simulink model "Fig330L1_THD5_tuned_gridRC2_2wai"  (R2021b)
settings: Solver=ode45  StartTime=0.0  StopTime=0.3  RelTol=1e-3
libraries: spsSeriesRLCBranchLib x17, spsThreePhaseVIMeasurementLib x6, spsIGBTDiodeLib x6, spsGroundLib x4, eePowerMeasurement x4, spsVoltageMeasurementLib x4, spsSecondOrderFilterLib x2, spsabctoAlphaBetaZeroLib x2, spsabctodq0Lib x2, spsDCVoltageSourceLib x1, simulink x1, spsThreePhaseProgrammableVoltageSourceLib x1
settings Model: Creator=cym1999  LastModifiedBy=caoyanmin
settings DataIOCC: ReturnWorkspaceOutputs=off

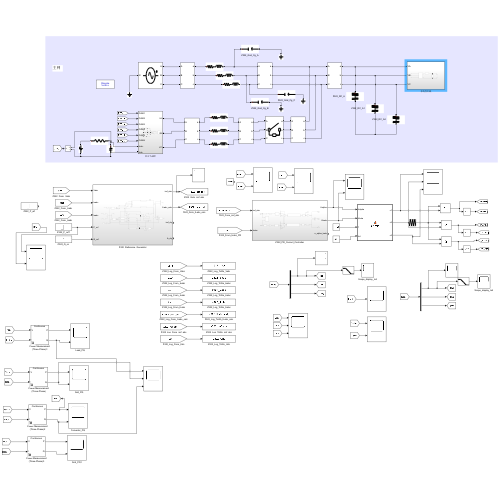
[thumbnail: Simulink's stored preview of the top-level diagram]
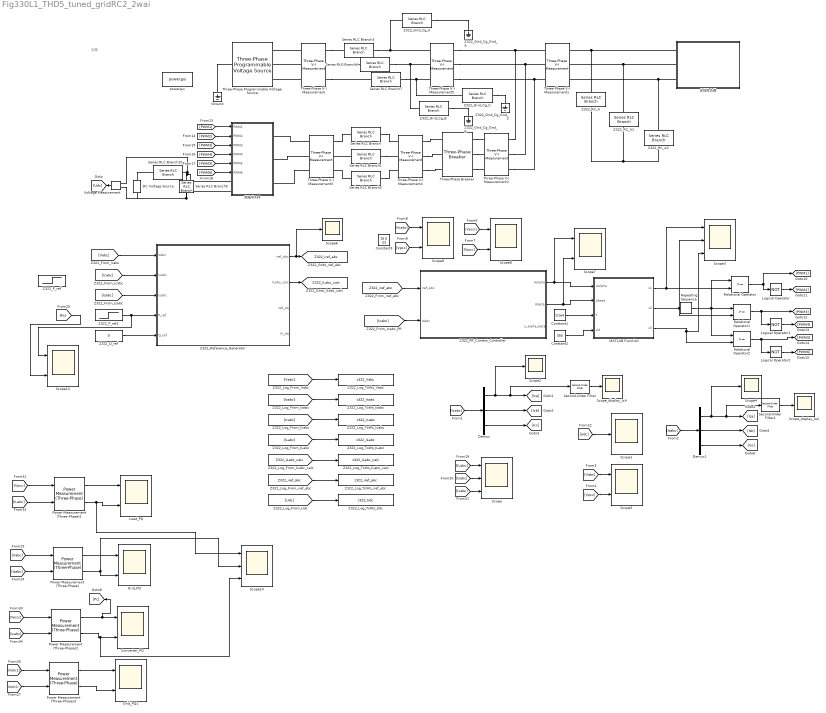
== system Fig330L1_THD5_tuned_gridRC2_2wai ==
  note: 主网
  Constant1 : Constant  Value=1/1e4
  Constant2 : Constant  Value=350
  Constant3 : Constant  Value=[0 0 0]
  Converter_PQ : Scope  NumInputPorts=2
  DC Voltage Source : spsDCVoltageSourceLib/DC Voltage Source  Amplitude=350  Measurements=None
  Demux : Demux  Outputs=3
  Demux1 : Demux  Outputs=3
  Grid_PQ : Scope  NumInputPorts=2
  Grid_PQ1 : Scope  NumInputPorts=2
  Ground : spsGroundLib/Ground  LConnTagsString=a
  Load_PQ : Scope  NumInputPorts=2
  Logical Operator : Logic  Operator=NOT  Inputs=1  AllPortsSameDT=off  OutDataTypeStr=boolean
  Logical Operator1 : Logic  Operator=NOT  Inputs=1  AllPortsSameDT=off  OutDataTypeStr=boolean
  Logical Operator2 : Logic  Operator=NOT  Inputs=1  AllPortsSameDT=off  OutDataTypeStr=boolean
  MATLAB Function : MATLAB Function  TreatAsAtomicUnit=on
  Power Measurement (Three-Phase){,1..3} (4 alike) : eePowerMeasurement/Power Measurement (Three-Phase)  LabelModeActiveChoice=Continuous  F=50  K=[1]  Seq=Positive  Ts=0
      settings: SourceProductBaseCode=PS
  Relational Operator : RelationalOperator  OutDataTypeStr=boolean  RndMeth=Simplest
  Relational Operator1 : RelationalOperator  OutDataTypeStr=boolean  RndMeth=Simplest
  Relational Operator2 : RelationalOperator  OutDataTypeStr=boolean  RndMeth=Simplest
  Repeating Sequence : simulink/Sources/Repeating Sequence  rep_seq_t=[0 0.00005 0.0001]  rep_seq_y=[0 0.0001/2 0]
  Scope : Scope  NumInputPorts=3
  Scope{1..2,4,6} (4 alike) : Scope
  Scope{5,7..9,13} (5 alike) : Scope  NumInputPorts=2
  Scope14 : Scope  NumInputPorts=3
  Scope3 : Scope  NumInputPorts=3
  Scope_display_IcA : Scope
  Scope_display_IsA : Scope
  Second-Order Filter : spsSecondOrderFilterLib/Second-Order Filter  FilterType=Lowpass  Fo=1000  Zeta=0.707  Ts=1e-6  Initialize=on  Vac_Init="[0,  0,  60]"  Vdc_Init=0  PlotResponse=off  FreqRange=[0, 500, 1]
      settings: SourceProductBaseCode=PS
  Second-Order Filter1 : spsSecondOrderFilterLib/Second-Order Filter  FilterType=Lowpass  Fo=1000  Zeta=0.707  Ts=1e-6  Initialize=on  Vac_Init="[0,  0,  60]"  Vdc_Init=0  PlotResponse=off  FreqRange=[0, 500, 1]
      settings: SourceProductBaseCode=PS
  Series RLC Branch : spsSeriesRLCBranchLib/Series RLC Branch  LConnTagsString=__new0  RConnTagsString=__new0  BranchType=RL  Resistance=0.05  Inductance=5e-4  SetiL0=off  InitialCurrent=0  Capacitance=1e-6  Setx0=off  InitialVoltage=0  Measurements=None
  Series RLC Branch1 : spsSeriesRLCBranchLib/Series RLC Branch  LConnTagsString=__new0  RConnTagsString=__new0  BranchType=RL  Resistance=0.05  Inductance=5e-4  SetiL0=off  InitialCurrent=0  Capacitance=1e-6  Setx0=off  InitialVoltage=0  Measurements=None
  Series RLC Branch10 : spsSeriesRLCBranchLib/Series RLC Branch  LConnTagsString=__new0  RConnTagsString=__new0  BranchType=R  Resistance=0.01  Inductance=2.56e-3  SetiL0=off  InitialCurrent=0  Capacitance=1e-6  Setx0=off  InitialVoltage=0  Measurements=None
  Series RLC Branch2 : spsSeriesRLCBranchLib/Series RLC Branch  LConnTagsString=__new0  RConnTagsString=__new0  BranchType=RL  Resistance=0.05  Inductance=5e-4  SetiL0=off  InitialCurrent=0  Capacitance=1e-6  Setx0=off  InitialVoltage=0  Measurements=None
  Series RLC Branch3 : spsSeriesRLCBranchLib/Series RLC Branch  LConnTagsString=__new0  RConnTagsString=__new0  BranchType=RL  Resistance=0.5  Inductance=3e-3  SetiL0=off  InitialCurrent=0  Capacitance=1e-6  Setx0=off  InitialVoltage=0  Measurements=None
  Series RLC Branch6 : spsSeriesRLCBranchLib/Series RLC Branch  LConnTagsString=__new0  RConnTagsString=__new0  BranchType=RL  Resistance=0.5  Inductance=3e-3  SetiL0=off  InitialCurrent=0  Capacitance=1e-6  Setx0=off  InitialVoltage=0  Measurements=None
  Series RLC Branch7 : spsSeriesRLCBranchLib/Series RLC Branch  LConnTagsString=__new0  RConnTagsString=__new0  BranchType=RL  Resistance=0.5  Inductance=3e-3  SetiL0=off  InitialCurrent=0  Capacitance=1e-6  Setx0=off  InitialVoltage=0  Measurements=None
  Series RLC Branch9 : spsSeriesRLCBranchLib/Series RLC Branch  LConnTagsString=__new0  RConnTagsString=__new0  BranchType=C  Resistance=0.05  Inductance=2.56e-4  SetiL0=off  InitialCurrent=0  Capacitance=0.0044  Setx0=off  InitialVoltage=800  Measurements=None
  Three-Phase Programmable Voltage Source : spsThreePhaseProgrammableVoltageSourceLib/Three-Phase Programmable Voltage Source  PositiveSequence=[110 0 50]  VariationEntity=None  VariationType=Table of time-amplitude pairs  VariationTypeAlt=Step  VariationStep=0.5  VariationRate=10  VariationMagnitude=0.3  VariationFrequency=2  VariationTiming=[1 2]  VariationPhaseA=off  Amplitudes=[1 0.8 1.2 1.0]  TimeValues=[0 0.1 0.15 0.2]  HarmonicGeneration=off  HarmonicA=[3 0.2 -25 0]  HarmonicB=[2 0.15 35 2]  Timing="[0.05  3]"  BusType=swing  Pref=0  Qref=0  Qmin=-inf  Qmax=inf
  Three-Phase V-I Measurement : spsThreePhaseVIMeasurementLib/Three-Phase V-I Measurement  VoltageMeasurement=phase-to-ground  SetLabelV=on  LabelV=Vabc  Vpu=off  VpuLL=off  CurrentMeasurement=yes  SetLabelI=on  LabelI=Isabc  Ipu=off  Pbase=100e6  Vbase=500e3  OutputType=Complex  PhasorSimulation=off  PSBequivalent=0
  Three-Phase V-I Measurement1 : spsThreePhaseVIMeasurementLib/Three-Phase V-I Measurement  VoltageMeasurement=phase-to-ground  SetLabelV=on  LabelV=Vpcc  Vpu=off  VpuLL=off  CurrentMeasurement=yes  SetLabelI=on  LabelI=ILabc  Ipu=off  Pbase=100e6  Vbase=500e3  OutputType=Complex  PhasorSimulation=off  PSBequivalent=0
  Three-Phase V-I Measurement2 : spsThreePhaseVIMeasurementLib/Three-Phase V-I Measurement  VoltageMeasurement=phase-to-ground  SetLabelV=on  LabelV=Vpccc  Vpu=off  VpuLL=off  CurrentMeasurement=yes  SetLabelI=on  LabelI=Icabc  Ipu=off  Pbase=100e6  Vbase=500e3  OutputType=Complex  PhasorSimulation=off  PSBequivalent=0
  Three-Phase V-I Measurement3 : spsThreePhaseVIMeasurementLib/Three-Phase V-I Measurement  VoltageMeasurement=no  SetLabelV=off  LabelV=Vinvabc  Vpu=on  VpuLL=off  CurrentMeasurement=yes  SetLabelI=on  LabelI=Iabc  Ipu=off  Pbase=100e6  Vbase=500e3  OutputType=Complex  PhasorSimulation=off  PSBequivalent=0
  Three-Phase V-I Measurement4 : spsThreePhaseVIMeasurementLib/Three-Phase V-I Measurement  VoltageMeasurement=phase-to-ground  SetLabelV=on  LabelV=Vcabc  Vpu=off  VpuLL=off  CurrentMeasurement=no  SetLabelI=off  LabelI=Icabc  Ipu=off  Pbase=100e6  Vbase=500e3  OutputType=Complex  PhasorSimulation=off  PSBequivalent=0
  Three-Phase V-I Measurement5 : spsThreePhaseVIMeasurementLib/Three-Phase V-I Measurement  VoltageMeasurement=phase-to-ground  SetLabelV=on  LabelV=Vabc1  Vpu=off  VpuLL=off  CurrentMeasurement=yes  SetLabelI=on  LabelI=Isabc1  Ipu=off  Pbase=100e6  Vbase=500e3  OutputType=Complex  PhasorSimulation=off  PSBequivalent=0
  Three-Phase Breaker : spsThreePhaseBreakerLib/Three-Phase Breaker  InitialState=open  SwitchA=on  SwitchB=on  SwitchC=on  SwitchTimes=[0.1]  External=off  BreakerResistance=0.01  SnubberResistance=1e8  SnubberCapacitance=inf  Measurements=None
  Voltage Measurement : spsVoltageMeasurementLib/Voltage Measurement  PhasorSimulation=off  OutputType=Complex  PSBequivalent=0
  Z322_Grid_Cg_A : spsSeriesRLCBranchLib/Series RLC Branch  LConnTagsString=__new0  RConnTagsString=__new0  BranchType=C  Resistance=0.3  Inductance=3e-3  SetiL0=off  InitialCurrent=0  Capacitance=20e-6  Setx0=off  InitialVoltage=0  Measurements=None
  Z322_Grid_Cg_B : spsSeriesRLCBranchLib/Series RLC Branch  LConnTagsString=__new0  RConnTagsString=__new0  BranchType=C  Resistance=0.3  Inductance=3e-3  SetiL0=off  InitialCurrent=0  Capacitance=20e-6  Setx0=off  InitialVoltage=0  Measurements=None
  Z322_Grid_Cg_C : spsSeriesRLCBranchLib/Series RLC Branch  LConnTagsString=__new0  RConnTagsString=__new0  BranchType=C  Resistance=0.3  Inductance=3e-3  SetiL0=off  InitialCurrent=0  Capacitance=20e-6  Setx0=off  InitialVoltage=0  Measurements=None
  Z322_Grid_Cg_Gnd_A : spsGroundLib/Ground  LConnTagsString=a
  Z322_Grid_Cg_Gnd_B : spsGroundLib/Ground  LConnTagsString=a
  Z322_Grid_Cg_Gnd_C : spsGroundLib/Ground  LConnTagsString=a
  Z322_Log_ToWs_ILabc : ToWorkspace  VariableName=z322_ILabc  SaveFormat=Structure With Time  SampleTime=-1
  Z322_Log_ToWs_ILabc_calc : ToWorkspace  VariableName=z322_ILabc_calc  SaveFormat=Structure With Time  SampleTime=-1
  Z322_Log_ToWs_Icabc : ToWorkspace  VariableName=z322_Icabc  SaveFormat=Structure With Time  SampleTime=-1
  Z322_Log_ToWs_Isabc : ToWorkspace  VariableName=z322_Isabc  SaveFormat=Structure With Time  SampleTime=-1
  Z322_Log_ToWs_Udc : ToWorkspace  VariableName=z322_Udc  SaveFormat=Structure With Time  SampleTime=-1
  Z322_Log_ToWs_Vabc : ToWorkspace  VariableName=z322_Vabc  SaveFormat=Structure With Time  SampleTime=-1
  Z322_Log_ToWs_iref_abc : ToWorkspace  VariableName=z322_iref_abc  SaveFormat=Structure With Time  SampleTime=-1
  Z322_PR_Current_Controller : Subsystem
  Z322_P_ref : Step  Time=0.3  Before=5000  After=8000  SampleTime=0
  Z322_P_ref1 : Step  Time=0.1  Before=5000  After=8000  SampleTime=0
  Z322_Q_ref : Constant  Value=0
  Z322_RC_A : spsSeriesRLCBranchLib/Series RLC Branch  LConnTagsString=__new0  RConnTagsString=__new0  BranchType=RC  Resistance=10  Inductance=2.56e-4  SetiL0=off  InitialCurrent=0  Capacitance=1e-3  Setx0=off  InitialVoltage=220  Measurements=None
  Z322_RC_A1 : spsSeriesRLCBranchLib/Series RLC Branch  LConnTagsString=__new0  RConnTagsString=__new0  BranchType=RC  Resistance=10  Inductance=2.56e-4  SetiL0=off  InitialCurrent=0  Capacitance=1e-3  Setx0=off  InitialVoltage=220  Measurements=None
  Z322_RC_A2 : spsSeriesRLCBranchLib/Series RLC Branch  LConnTagsString=__new0  RConnTagsString=__new0  BranchType=RC  Resistance=10  Inductance=2.56e-4  SetiL0=off  InitialCurrent=0  Capacitance=1e-3  Setx0=off  InitialVoltage=220  Measurements=None
  Z322_Reference_Generator : Subsystem
  powergui : spspowerguiLib/powergui  Priority=1  SimulationMode=Discrete  SampleTime=1e-6  frequency=60  Iterations=50  frequencyindice=50  Pbase=100e6  ErrMax=1e-4  UnitsV=kV  UnitsW=MW  buscounter=0  FunctionMessages=off  echomessages=off  EnableUseOfTLC=off  CurrentSourceSwitches=off  DisableSnubberDevices=off  DisableRonSwitches=off  DisableVfSwitches=off  DisplayEquations=off  AutomaticDiscreteSolvers=off  SolverType=Tustin/Backward Euler (TBE)  Interpol=off  ExternalGateDelay=off  methode=off  Ts=100  x0status=blocks  SPID=on  SwTol=0  HookPort=off  NonlinearTolerance=1e-4  nMaxIteration=100  ContinueOnMaxIteration=off  RestoreLinks=warning  ResistiveCurrentMeasurement=off  Frange=[0:2:500]  Ylog=off  Xlog=on  ShowGrid=off  save=off  variable=ZData  structure=0  ZoomFFT=off  StartTime=0.0  cycles=1  DisplayStyle=1  fundamental=60  FreqAxis=off  MaxFrequency=1000  frequencyindicesteady=1  RmsSteady=1  display=off
  两电平APF : Subsystem
  非线性负载 : Subsystem
  tag scope: Z322_ILabc_calc=global, Z322_iref_abc=global
  wires:
  Constant1/1 -> MATLAB Function/3(T)
  Constant2/1 -> MATLAB Function/4(Ud)
  Relational Operator/1 -> Logical Operator/1, [PWM1]
  Relational Operator1/1 -> [PWM3], Logical Operator1/1
  Relational Operator2/1 -> [PWM5], Logical Operator2/1
  Logical Operator/1 -> [PWM2]
  Logical Operator1/1 -> [PWM4]
  Logical Operator2/1 -> [PWM6]
  [PWM1] -> 两电平APF/1(PWM1)
  [PWM2] -> 两电平APF/2(PWM2)
  [PWM3] -> 两电平APF/3(PWM3)
  [PWM4] -> 两电平APF/4(PWM4)
  [PWM5] -> 两电平APF/5(PWM5)
  [PWM6] -> 两电平APF/6(PWM6)
  [ILabc] -> Scope/1
  [Isabc] -> Scope/2
  [Icabc] -> Scope/3
  [Udc] -> Scope1/1
  [Vabc] -> Power Measurement (Three-Phase)/1
  [Isabc] -> Power Measurement (Three-Phase)/2
  Power Measurement (Three-Phase)/1 -> Grid_PQ/1
  Power Measurement (Three-Phase)/2 -> Grid_PQ/2, Scope14/2
  Repeating Sequence/1 -> Relational Operator2/1, Relational Operator/1, Relational Operator1/1
  MATLAB Function/1(c1) -> Relational Operator/2, Scope3/1
  MATLAB Function/2(c2) -> Relational Operator1/2, Scope3/2
  MATLAB Function/3(c3) -> Relational Operator2/2, Scope3/3
  [ILabc] -> Power Measurement (Three-Phase)1/2
  Power Measurement (Three-Phase)1/1 -> Load_PQ/1
  [Vpcc] -> Power Measurement (Three-Phase)1/1
  Power Measurement (Three-Phase)1/2 -> Scope14/1, Load_PQ/2
  [Icabc] -> Power Measurement (Three-Phase)2/2
  Power Measurement (Three-Phase)2/1 -> [Pc], Converter_PQ/1
  [Vpccc] -> Power Measurement (Three-Phase)2/1
  Power Measurement (Three-Phase)2/2 -> Scope14/3, Converter_PQ/2
  Voltage Measurement/1 -> [Udc]
  [Vabc] -> Z322_Reference_Generator/1(Vabc)
  [Icabc] -> Z322_Reference_Generator/2(Icabc)
  [Isabc] -> Z322_Reference_Generator/3(Isabc)
  Z322_P_ref1/1 -> Scope13/1, Z322_Reference_Generator/4(P_ref)
  Z322_Q_ref/1 -> Z322_Reference_Generator/5(Q_ref)
  Z322_Reference_Generator/1(iref_abc) -> Scope6/1, [Z322_iref_abc]
  Z322_Reference_Generator/2(ILabc_calc) -> [Z322_ILabc_calc]
  [Icabc] -> Z322_PR_Current_Controller/2(Icabc)
  [Vabc] -> Z322_Log_ToWs_Vabc/1
  [Isabc] -> Z322_Log_ToWs_Isabc/1
  [Icabc] -> Z322_Log_ToWs_Icabc/1
  [ILabc] -> Z322_Log_ToWs_ILabc/1
  [Z322_ILabc_calc] -> Z322_Log_ToWs_ILabc_calc/1
  [Z322_iref_abc] -> Z322_Log_ToWs_iref_abc/1
  [Udc] -> Z322_Log_ToWs_Udc/1
  [Icabc] -> Demux/1
  Demux/1 -> Scope2/1, Second-Order Filter/1, [Ica]
  Demux/2 -> [Icb]
  Demux/3 -> [Icc]
  Second-Order Filter/1 -> Scope_display_IcA/1
  Second-Order Filter1/1 -> Scope_display_IsA/1
  [Isabc] -> Demux1/1
  Demux1/1 -> Scope4/1, Second-Order Filter1/1, [Isa]
  Demux1/2 -> [Isb]
  Demux1/3 -> [Isc]
  [Vabc] -> Scope5/1
  [Vpcc] -> Scope5/2
  Z322_PR_Current_Controller/1(Ualpha) -> Scope7/1, MATLAB Function/1(Ualpha)
  Z322_PR_Current_Controller/2(Ubeta) -> Scope7/2, MATLAB Function/2(Ubeta)
  [Z322_iref_abc] -> Z322_PR_Current_Controller/1(iref_abc)
  [Vpccc] -> Scope8/1
  [Vpcc] -> Scope8/2
  [Vpcc] -> Scope9/2
  [Vcabc] -> Scope9/1
  [Pc] -> Scope13/2
  [Vabc1] -> Power Measurement (Three-Phase)3/1
  Power Measurement (Three-Phase)3/2 -> Grid_PQ1/2
  [Isabc1] -> Power Measurement (Three-Phase)3/2
  Power Measurement (Three-Phase)3/1 -> Grid_PQ1/1
  connections:
  Three-Phase Programmable Voltage Source/LConn1 -- Ground/LConn1
  Three-Phase V-I Measurement/LConn1 -- Three-Phase Programmable Voltage Source/RConn1
  Three-Phase V-I Measurement/LConn2 -- Three-Phase Programmable Voltage Source/RConn2
  Three-Phase V-I Measurement/LConn3 -- Three-Phase Programmable Voltage Source/RConn3
  Three-Phase V-I Measurement2/RConn1 -- Three-Phase V-I Measurement5/RConn1 -- Three-Phase V-I Measurement1/LConn1
  Three-Phase V-I Measurement2/RConn2 -- Three-Phase V-I Measurement1/LConn2 -- Three-Phase V-I Measurement5/RConn2
  Three-Phase V-I Measurement2/RConn3 -- Three-Phase V-I Measurement1/LConn3 -- Three-Phase V-I Measurement5/RConn3
  非线性负载/LConn1 -- Three-Phase V-I Measurement1/RConn1 -- Z322_RC_A/LConn1
  非线性负载/LConn2 -- Z322_RC_A1/LConn1 -- Three-Phase V-I Measurement1/RConn2
  非线性负载/LConn3 -- Three-Phase V-I Measurement1/RConn3 -- Z322_RC_A2/LConn1
  Three-Phase Breaker/RConn2 -- Three-Phase V-I Measurement2/LConn2
  Three-Phase Breaker/RConn1 -- Three-Phase V-I Measurement2/LConn1
  Three-Phase Breaker/RConn3 -- Three-Phase V-I Measurement2/LConn3
  Three-Phase V-I Measurement3/RConn1 -- Series RLC Branch/LConn1
  Series RLC Branch1/LConn1 -- Three-Phase V-I Measurement3/RConn2
  Series RLC Branch2/LConn1 -- Three-Phase V-I Measurement3/RConn3
  Three-Phase V-I Measurement3/LConn1 -- 两电平APF/RConn1
  Three-Phase V-I Measurement3/LConn2 -- 两电平APF/RConn2
  Three-Phase V-I Measurement3/LConn3 -- 两电平APF/RConn3
  DC Voltage Source/RConn1 -- Series RLC Branch10/LConn1
  Series RLC Branch9/RConn1 -- DC Voltage Source/LConn1 -- Voltage Measurement/LConn2 -- 两电平APF/LConn2
  Series RLC Branch10/RConn1 -- Series RLC Branch9/LConn1 -- 两电平APF/LConn1 -- Voltage Measurement/LConn1
  Z322_RC_A/RConn1 -- Z322_RC_A2/RConn1 -- Z322_RC_A1/RConn1
  Three-Phase V-I Measurement/RConn1 -- Series RLC Branch3/LConn1
  Three-Phase V-I Measurement/RConn2 -- Series RLC Branch6/LConn1
  Three-Phase V-I Measurement/RConn3 -- Series RLC Branch7/LConn1
  Series RLC Branch2/RConn1 -- Three-Phase V-I Measurement4/LConn3
  Series RLC Branch1/RConn1 -- Three-Phase V-I Measurement4/LConn2
  Series RLC Branch/RConn1 -- Three-Phase V-I Measurement4/LConn1
  Three-Phase V-I Measurement4/RConn1 -- Three-Phase Breaker/LConn1
  Three-Phase V-I Measurement4/RConn2 -- Three-Phase Breaker/LConn2
  Three-Phase V-I Measurement4/RConn3 -- Three-Phase Breaker/LConn3
  Series RLC Branch3/RConn1 -- Three-Phase V-I Measurement5/LConn1 -- Z322_Grid_Cg_A/LConn1
  Series RLC Branch6/RConn1 -- Three-Phase V-I Measurement5/LConn2 -- Z322_Grid_Cg_B/LConn1
  Series RLC Branch7/RConn1 -- Three-Phase V-I Measurement5/LConn3 -- Z322_Grid_Cg_C/LConn1
  Z322_Grid_Cg_A/RConn1 -- Z322_Grid_Cg_Gnd_A/LConn1
  Z322_Grid_Cg_B/RConn1 -- Z322_Grid_Cg_Gnd_B/LConn1
  Z322_Grid_Cg_C/RConn1 -- Z322_Grid_Cg_Gnd_C/LConn1

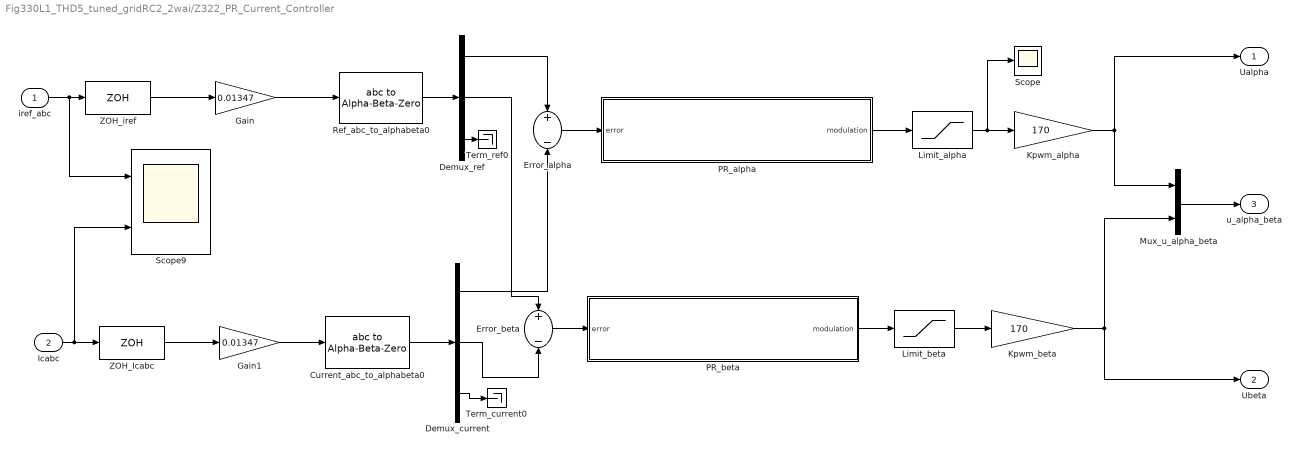
== system Fig330L1_THD5_tuned_gridRC2_2wai/Z322_PR_Current_Controller ==
  iref_abc : Inport
  Icabc : Inport  Port=2
  Current_abc_to_alphabeta0 : spsabctoAlphaBetaZeroLib/abc to Alpha-Beta-Zero
      settings: SourceProductBaseCode=PS
  Demux_current : Demux  Outputs=3
  Demux_ref : Demux  Outputs=3
  Error_alpha : Sum  Inputs=+-
  Error_beta : Sum  Inputs=+-
  Gain : Gain  Gain=0.01347
  Gain1 : Gain  Gain=0.01347
  Kpwm_alpha : Gain  Gain=170
  Kpwm_beta : Gain  Gain=170
  Limit_alpha : Saturate  UpperLimit=0.95  LowerLimit=-0.95
  Limit_beta : Saturate  UpperLimit=0.95  LowerLimit=-0.95
  Mux_u_alpha_beta : Mux  Inputs=2
  PR_alpha : Subsystem
  PR_beta : Subsystem
  Ref_abc_to_alphabeta0 : spsabctoAlphaBetaZeroLib/abc to Alpha-Beta-Zero
      settings: SourceProductBaseCode=PS
  Scope : Scope
  Scope9 : Scope  NumInputPorts=2
  Term_current0 : Terminator
  Term_ref0 : Terminator
  ZOH_Icabc : ZeroOrderHold  SampleTime=5e-5
  ZOH_iref : ZeroOrderHold  SampleTime=5e-5
  Ualpha : Outport
  Ubeta : Outport  Port=2
  u_alpha_beta : Outport  Port=3
  wires:
  Icabc/1 -> Scope9/2, ZOH_Icabc/1
  Ref_abc_to_alphabeta0/1 -> Demux_ref/1
  Current_abc_to_alphabeta0/1 -> Demux_current/1
  Demux_ref/1 -> Error_alpha/1
  Demux_current/1 -> Error_alpha/2
  Demux_ref/2 -> Error_beta/1
  Demux_current/2 -> Error_beta/2
  Demux_ref/3 -> Term_ref0/1
  Demux_current/3 -> Term_current0/1
  Error_alpha/1 -> PR_alpha/1(error)
  Error_beta/1 -> PR_beta/1(error)
  PR_alpha/1(modulation) -> Limit_alpha/1
  PR_beta/1(modulation) -> Limit_beta/1
  Limit_alpha/1 -> Scope/1, Kpwm_alpha/1
  Limit_beta/1 -> Kpwm_beta/1
  Kpwm_alpha/1 -> Ualpha/1, Mux_u_alpha_beta/1
  Kpwm_beta/1 -> Mux_u_alpha_beta/2, Ubeta/1
  Mux_u_alpha_beta/1 -> u_alpha_beta/1
  ZOH_iref/1 -> Gain/1
  Gain/1 -> Ref_abc_to_alphabeta0/1
  ZOH_Icabc/1 -> Gain1/1
  Gain1/1 -> Current_abc_to_alphabeta0/1
  iref_abc/1 -> Scope9/1, ZOH_iref/1

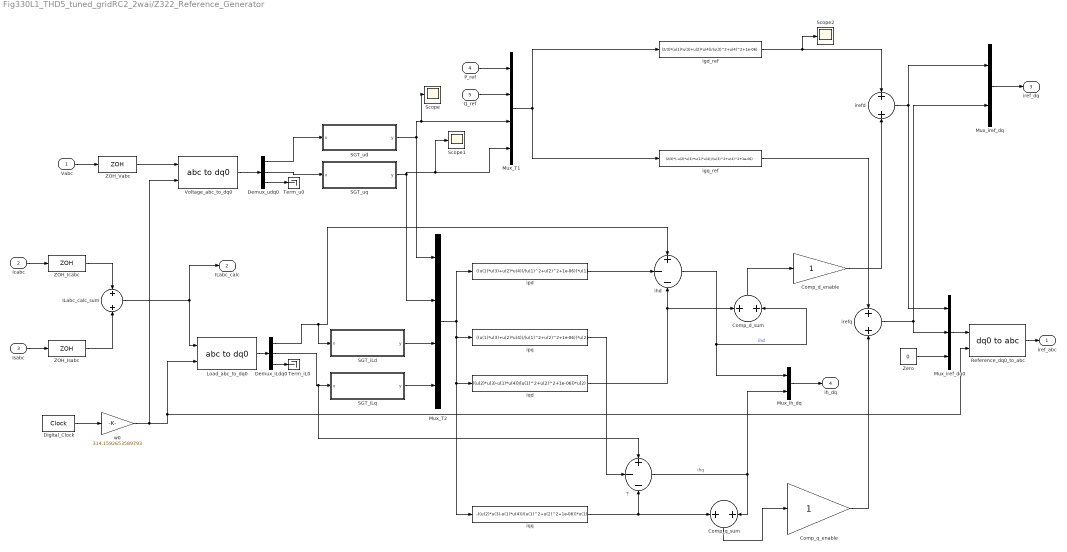
== system Fig330L1_THD5_tuned_gridRC2_2wai/Z322_Reference_Generator ==
  Vabc : Inport
  Icabc : Inport  Port=2
  Isabc : Inport  Port=3
  P_ref : Inport  Port=4
  Q_ref : Inport  Port=5
  Comp_d_enable : Gain
  Comp_d_sum : Sum
  Comp_q_enable : Gain
  Comp_q_sum : Sum
  Demux_iLdq0 : Demux  Outputs=3
  Demux_udq0 : Demux  Outputs=3
  Digital_Clock : DigitalClock  SampleTime=5e-5
  ILabc_calc_sum : Sum
  Load_abc_to_dq0 : spsabctodq0Lib/abc to dq0  Alignment=90 degrees behind phase A axis
  Mux_T1 : Mux
  Mux_T2 : Mux
  Mux_ih_dq : Mux  Inputs=2
  Mux_iref_dq : Mux  Inputs=2
  Mux_iref_dq0 : Mux  Inputs=3
  Reference_dq0_to_abc : spsdq0toabcLib/dq0 to abc  Alignment=90 degrees behind phase A axis
  SGT_iLd : Subsystem
  SGT_iLq : Subsystem
  SGT_ud : Subsystem
  SGT_uq : Subsystem
  Scope : Scope
  Scope1 : Scope
  Scope2 : Scope
  Term_iL0 : Terminator
  Term_u0 : Terminator
  Voltage_abc_to_dq0 : spsabctodq0Lib/abc to dq0  Alignment=90 degrees behind phase A axis
  ZOH_Icabc : ZeroOrderHold  SampleTime=5e-5
  ZOH_Isabc : ZeroOrderHold  SampleTime=5e-5
  ZOH_Vabc : ZeroOrderHold  SampleTime=5e-5
  Zero : Constant  Value=0
  igd_ref : Fcn  Expr=(2/3)*(u(1)*u(3)+u(2)*u(4))/(u(3)^2+u(4)^2+1e-06)
  igq_ref : Fcn  Expr=(2/3)*(-u(2)*u(3)+u(1)*u(4))/(u(3)^2+u(4)^2+1e-06)
  ihd : Sum  Inputs=+--
  ipd : Fcn  Expr=((u(1)*u(3)+u(2)*u(4))/(u(1)^2+u(2)^2+1e-06))*u(1)
  ipq : Fcn  Expr=((u(1)*u(3)+u(2)*u(4))/(u(1)^2+u(2)^2+1e-06))*u(2)
  iqd : Fcn  Expr=((u(2)*u(3)-u(1)*u(4))/(u(1)^2+u(2)^2+1e-06))*u(2)
  iqq : Fcn  Expr=-((u(2)*u(3)-u(1)*u(4))/(u(1)^2+u(2)^2+1e-06))*u(1)
  irefd : Sum
  irefq : Sum
  w0 : Gain  Gain=314.1592653589793
  ？ : Sum  Inputs=+--
  iref_abc : Outport
  ILabc_calc : Outport  Port=2
  iref_dq : Outport  Port=3
  ih_dq : Outport  Port=4
  wires:
  Vabc/1 -> ZOH_Vabc/1
  Icabc/1 -> ZOH_Icabc/1
  Isabc/1 -> ZOH_Isabc/1
  ZOH_Icabc/1 -> ILabc_calc_sum/1
  ZOH_Isabc/1 -> ILabc_calc_sum/2
  ILabc_calc_sum/1 -> Load_abc_to_dq0/1, ILabc_calc/1
  Digital_Clock/1 -> w0/1
  ZOH_Vabc/1 -> Voltage_abc_to_dq0/1
  w0/1 -> Voltage_abc_to_dq0/2, Load_abc_to_dq0/2, Reference_dq0_to_abc/2
  Voltage_abc_to_dq0/1 -> Demux_udq0/1
  Load_abc_to_dq0/1 -> Demux_iLdq0/1
  Demux_udq0/1 -> SGT_ud/1(x)
  Demux_udq0/2 -> SGT_uq/1(x)
  Demux_iLdq0/1 -> ihd/1, SGT_iLd/1(x)
  Demux_iLdq0/2 -> ？/1, SGT_iLq/1(x)
  Demux_udq0/3 -> Term_u0/1
  Demux_iLdq0/3 -> Term_iL0/1
  P_ref/1 -> Mux_T1/1
  Q_ref/1 -> Mux_T1/2
  SGT_ud/1(y) -> Mux_T2/1, Scope/1, Mux_T1/3
  SGT_uq/1(y) -> Scope1/1, Mux_T1/4, Mux_T2/2
  SGT_iLd/1(y) -> Mux_T2/3
  SGT_iLq/1(y) -> Mux_T2/4
  Mux_T1/1 -> igq_ref/1, igd_ref/1
  Mux_T2/1 -> iqq/1, iqd/1, ipq/1, ipd/1
  ipd/1 -> ihd/2
  iqd/1 -> ihd/3, Comp_d_sum/1
  ipq/1 -> ？/2
  iqq/1 -> ？/3, Comp_q_sum/1
  ihd/1 -> Mux_ih_dq/1, Comp_d_sum/2  "ihd"
  ？/1 -> Comp_q_sum/2, Mux_ih_dq/2  "ihq"
  Comp_d_sum/1 -> Comp_d_enable/1
  Comp_q_sum/1 -> Comp_q_enable/1
  igd_ref/1 -> Scope2/1, irefd/1
  Comp_d_enable/1 -> irefd/2
  igq_ref/1 -> irefq/1
  Comp_q_enable/1 -> irefq/2
  irefd/1 -> Mux_iref_dq0/1, Mux_iref_dq/1
  irefq/1 -> Mux_iref_dq0/2, Mux_iref_dq/2
  Zero/1 -> Mux_iref_dq0/3
  Mux_iref_dq0/1 -> Reference_dq0_to_abc/1
  Reference_dq0_to_abc/1 -> iref_abc/1
  Mux_iref_dq/1 -> iref_dq/1
  Mux_ih_dq/1 -> ih_dq/1

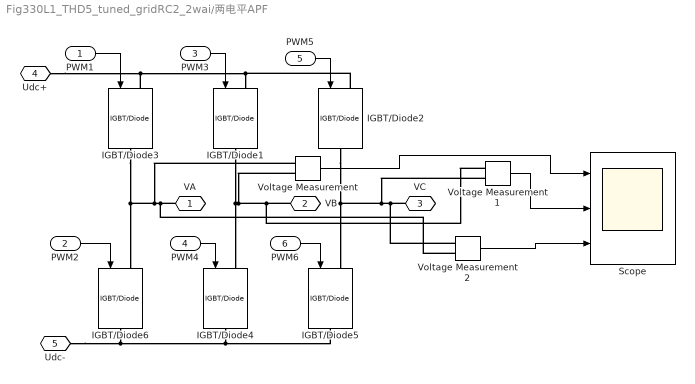
== system Fig330L1_THD5_tuned_gridRC2_2wai/两电平APF ==
  PWM1 : Inport
  PWM2 : Inport  Port=2
  PWM3 : Inport  Port=3
  PWM4 : Inport  Port=4
  PWM5 : Inport  Port=5
  PWM6 : Inport  Port=6
  IGBT/Diode{1..6} (6 alike) : spsIGBTDiodeLib/IGBT//Diode  Ron=1e-3  Rs=1e5  Cs=inf  Measurements=off
  Scope : Scope  NumInputPorts=3
  Voltage Measurement : spsVoltageMeasurementLib/Voltage Measurement  PhasorSimulation=off  OutputType=Complex  PSBequivalent=0
  Voltage Measurement1 : spsVoltageMeasurementLib/Voltage Measurement  PhasorSimulation=off  OutputType=Complex  PSBequivalent=0
  Voltage Measurement2 : spsVoltageMeasurementLib/Voltage Measurement  PhasorSimulation=off  OutputType=Complex  PSBequivalent=0
  VA : PMIOPort  Side=Right
  VB : PMIOPort  Port=2  Side=Right
  VC : PMIOPort  Port=3  Side=Right
  Udc+ : PMIOPort  Port=4  Side=Left
  Udc- : PMIOPort  Port=5  Side=Left
  wires:
  PWM3/1 -> IGBT/Diode1/1
  PWM4/1 -> IGBT/Diode4/1
  PWM2/1 -> IGBT/Diode6/1
  PWM6/1 -> IGBT/Diode5/1
  PWM1/1 -> IGBT/Diode3/1
  PWM5/1 -> IGBT/Diode2/1
  Voltage Measurement/1 -> Scope/1
  Voltage Measurement1/1 -> Scope/2
  Voltage Measurement2/1 -> Scope/3
  connections:
  IGBT/Diode3/LConn1 -- Udc+/RConn1 -- IGBT/Diode2/LConn1 -- IGBT/Diode1/LConn1
  IGBT/Diode3/RConn1 -- Voltage Measurement2/LConn2 -- VA/RConn1 -- Voltage Measurement/LConn1 -- IGBT/Diode6/LConn1
  IGBT/Diode2/RConn1 -- Voltage Measurement2/LConn1 -- VC/RConn1 -- Voltage Measurement1/LConn2 -- IGBT/Diode5/LConn1
  IGBT/Diode1/RConn1 -- Voltage Measurement1/LConn1 -- VB/RConn1 -- Voltage Measurement/LConn2 -- IGBT/Diode4/LConn1
  IGBT/Diode6/RConn1 -- Udc-/RConn1 -- IGBT/Diode4/RConn1 -- IGBT/Diode5/RConn1

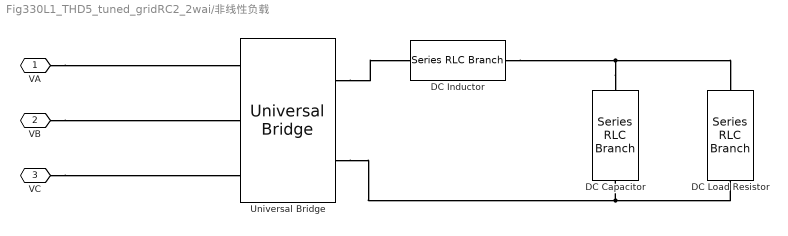
== system Fig330L1_THD5_tuned_gridRC2_2wai/非线性负载 ==
  DC Capacitor : spsSeriesRLCBranchLib/Series RLC Branch  LConnTagsString=__new0  RConnTagsString=__new0  BranchType=C  Resistance=1e-4  Inductance=1e-3  SetiL0=off  InitialCurrent=0  Capacitance=150e-06  Setx0=off  InitialVoltage=0  Measurements=None
  DC Inductor : spsSeriesRLCBranchLib/Series RLC Branch  LConnTagsString=__new0  RConnTagsString=__new0  BranchType=L  Resistance=1e-4  Inductance=1.5e-3  SetiL0=off  InitialCurrent=0  Capacitance=1e-6  Setx0=off  InitialVoltage=0  Measurements=None
  DC Load Resistor : spsSeriesRLCBranchLib/Series RLC Branch  LConnTagsString=__new0  RConnTagsString=__new0  BranchType=R  Resistance=20  Inductance=1e-3  SetiL0=off  InitialCurrent=0  Capacitance=1e-6  Setx0=off  InitialVoltage=0  Measurements=None
  Universal Bridge : spsUniversalBridgeLib/Universal Bridge  Arms=3  SnubberResistance=1e6  SnubberCapacitance=1e-12  Device=Diodes  Ron=1e-3  Lon=0  ForwardVoltages=[0 0]  ForwardVoltage=0  GTOparameters=[ 10e-6 , 20e-6 ]  IGBTparameters=[ 1e-6 , 2e-6 ]  Measurements=None  Measurements_2=None  converterType=Rectifier
  VA : PMIOPort  Side=Left
  VB : PMIOPort  Port=2  Side=Left
  VC : PMIOPort  Port=3  Side=Left
  connections:
  VA/RConn1 -- Universal Bridge/LConn1
  VB/RConn1 -- Universal Bridge/LConn2
  VC/RConn1 -- Universal Bridge/LConn3
  Universal Bridge/RConn1 -- DC Inductor/LConn1
  DC Capacitor/RConn1 -- DC Inductor/RConn1 -- DC Load Resistor/RConn1
  DC Capacitor/LConn1 -- Universal Bridge/RConn2 -- DC Load Resistor/LConn1

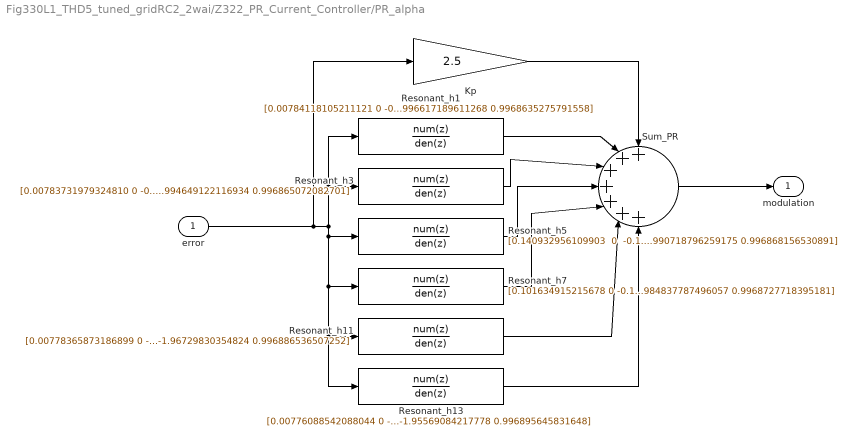
== system Fig330L1_THD5_tuned_gridRC2_2wai/Z322_PR_Current_Controller/PR_alpha ==
  error : Inport
  Kp : Gain  Gain=2.5
  Resonant_h1 : DiscreteTransferFcn  Numerator=[0.00784118105211121 0 -0.00784118105211121]  Denominator=[1 -1.996617189611268 0.9968635275791558]  SampleTime=5e-5
  Resonant_h11 : DiscreteTransferFcn  Numerator=[0.00778365873186899 0 -0.00778365873186899]  Denominator=[1 -1.96729830354824 0.996886536507252]  SampleTime=5e-5
  Resonant_h13 : DiscreteTransferFcn  Numerator=[0.00776088542088044 0 -0.00776088542088044]  Denominator=[1 -1.95569084217778 0.996895645831648]  SampleTime=5e-5
  Resonant_h3 : DiscreteTransferFcn  Numerator=[0.00783731979324810 0 -0.00783731979324810]  Denominator=[1 -1.994649122116934 0.996865072082701]  SampleTime=5e-5
  Resonant_h5 : DiscreteTransferFcn  Numerator="[0.140932956109903  0  -0.140932956109903]"  Denominator=[1 -1.990718796259175 0.996868156530891]  SampleTime=5e-5
  Resonant_h7 : DiscreteTransferFcn  Numerator=[0.101634915215678 0 -0.101634915215678]  Denominator=[1 -1.984837787496057 0.9968727718395181]  SampleTime=5e-5
  Sum_PR : Sum  Inputs=+++++++
  modulation : Outport
  wires:
  error/1 -> Resonant_h1/1, Resonant_h3/1, Resonant_h5/1, Resonant_h11/1, Resonant_h13/1, Resonant_h7/1, Kp/1
  Kp/1 -> Sum_PR/1
  Resonant_h1/1 -> Sum_PR/2
  Sum_PR/1 -> modulation/1
  Resonant_h13/1 -> Sum_PR/7
  Resonant_h11/1 -> Sum_PR/6
  Resonant_h7/1 -> Sum_PR/5
  Resonant_h5/1 -> Sum_PR/4
  Resonant_h3/1 -> Sum_PR/3

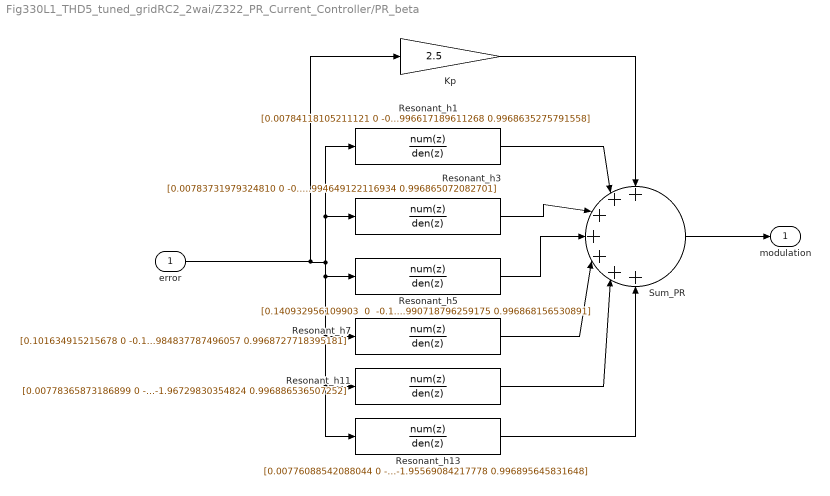
== system Fig330L1_THD5_tuned_gridRC2_2wai/Z322_PR_Current_Controller/PR_beta ==
  error : Inport
  Kp : Gain  Gain=2.5
  Resonant_h1 : DiscreteTransferFcn  Numerator=[0.00784118105211121 0 -0.00784118105211121]  Denominator=[1 -1.996617189611268 0.9968635275791558]  SampleTime=5e-5
  Resonant_h11 : DiscreteTransferFcn  Numerator=[0.00778365873186899 0 -0.00778365873186899]  Denominator=[1 -1.96729830354824 0.996886536507252]  SampleTime=5e-5
  Resonant_h13 : DiscreteTransferFcn  Numerator=[0.00776088542088044 0 -0.00776088542088044]  Denominator=[1 -1.95569084217778 0.996895645831648]  SampleTime=5e-5
  Resonant_h3 : DiscreteTransferFcn  Numerator=[0.00783731979324810 0 -0.00783731979324810]  Denominator=[1 -1.994649122116934 0.996865072082701]  SampleTime=5e-5
  Resonant_h5 : DiscreteTransferFcn  Numerator="[0.140932956109903  0  -0.140932956109903]"  Denominator=[1 -1.990718796259175 0.996868156530891]  SampleTime=5e-5
  Resonant_h7 : DiscreteTransferFcn  Numerator=[0.101634915215678 0 -0.101634915215678]  Denominator=[1 -1.984837787496057 0.9968727718395181]  SampleTime=5e-5
  Sum_PR : Sum  Inputs=+++++++
  modulation : Outport
  wires:
  error/1 -> Kp/1, Resonant_h1/1, Resonant_h3/1, Resonant_h13/1, Resonant_h11/1, Resonant_h7/1, Resonant_h5/1
  Kp/1 -> Sum_PR/1
  Resonant_h1/1 -> Sum_PR/2
  Resonant_h3/1 -> Sum_PR/3
  Resonant_h5/1 -> Sum_PR/4
  Sum_PR/1 -> modulation/1
  Resonant_h13/1 -> Sum_PR/7
  Resonant_h7/1 -> Sum_PR/5
  Resonant_h11/1 -> Sum_PR/6

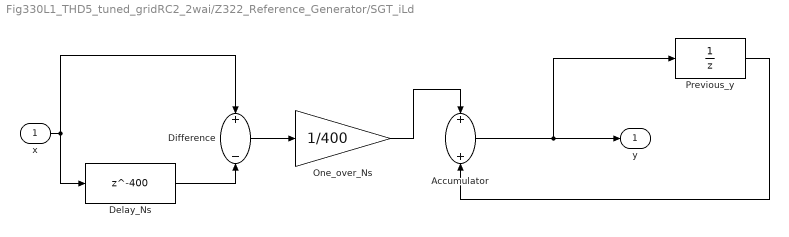
== system Fig330L1_THD5_tuned_gridRC2_2wai/Z322_Reference_Generator/SGT_iLd ==
  x : Inport
  Accumulator : Sum
  Delay_Ns : Delay  DelayLength=400  InitialCondition=0  SampleTime=5e-05
  Difference : Sum  Inputs=+-
  One_over_Ns : Gain  Gain=1/400
  Previous_y : UnitDelay  SampleTime=5e-05  HasFrameUpgradeWarning=on
  y : Outport
  wires:
  x/1 -> Delay_Ns/1, Difference/1
  Delay_Ns/1 -> Difference/2
  Difference/1 -> One_over_Ns/1
  One_over_Ns/1 -> Accumulator/1
  Previous_y/1 -> Accumulator/2
  Accumulator/1 -> Previous_y/1, y/1

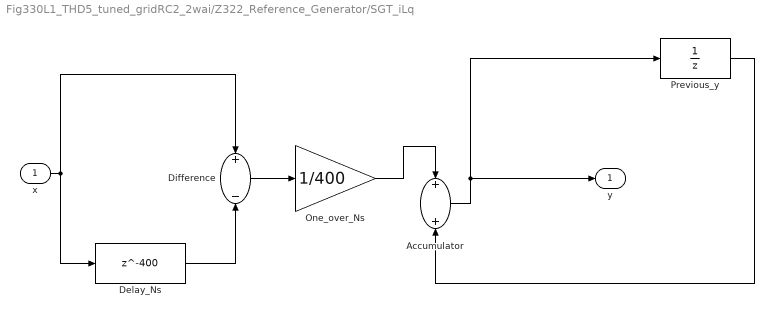
== system Fig330L1_THD5_tuned_gridRC2_2wai/Z322_Reference_Generator/SGT_iLq ==
  x : Inport
  Accumulator : Sum
  Delay_Ns : Delay  DelayLength=400  InitialCondition=0  SampleTime=5e-05
  Difference : Sum  Inputs=+-
  One_over_Ns : Gain  Gain=1/400
  Previous_y : UnitDelay  SampleTime=5e-05  HasFrameUpgradeWarning=on
  y : Outport
  wires:
  x/1 -> Delay_Ns/1, Difference/1
  Delay_Ns/1 -> Difference/2
  Difference/1 -> One_over_Ns/1
  One_over_Ns/1 -> Accumulator/1
  Previous_y/1 -> Accumulator/2
  Accumulator/1 -> Previous_y/1, y/1

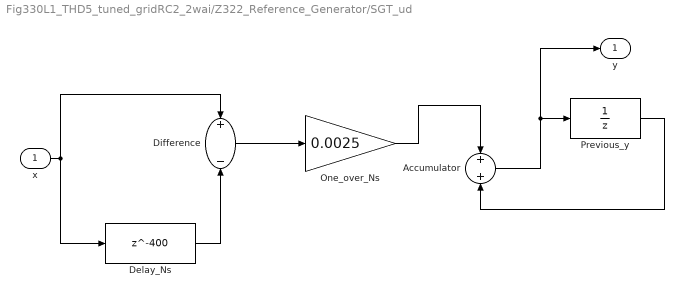
== system Fig330L1_THD5_tuned_gridRC2_2wai/Z322_Reference_Generator/SGT_ud ==
  x : Inport
  Accumulator : Sum
  Delay_Ns : Delay  DelayLength=400  InitialCondition=0  SampleTime=5e-05
  Difference : Sum  Inputs=+-
  One_over_Ns : Gain  Gain=0.0025
  Previous_y : UnitDelay  SampleTime=5e-5  HasFrameUpgradeWarning=on
  y : Outport
  wires:
  x/1 -> Delay_Ns/1, Difference/1
  Delay_Ns/1 -> Difference/2
  Difference/1 -> One_over_Ns/1
  One_over_Ns/1 -> Accumulator/1
  Previous_y/1 -> Accumulator/2
  Accumulator/1 -> y/1, Previous_y/1

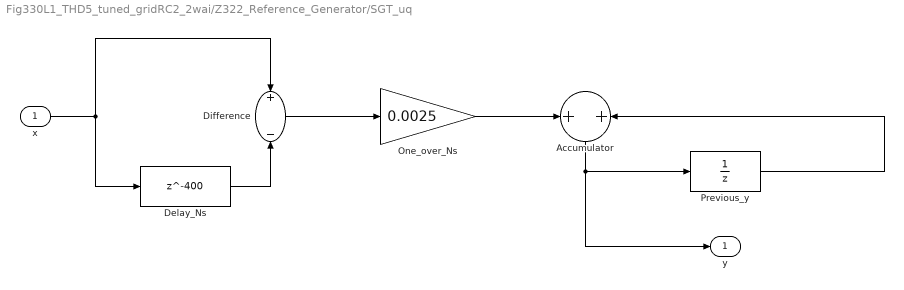
== system Fig330L1_THD5_tuned_gridRC2_2wai/Z322_Reference_Generator/SGT_uq ==
  x : Inport
  Accumulator : Sum
  Delay_Ns : Delay  DelayLength=400  InitialCondition=0  SampleTime=5e-05
  Difference : Sum  Inputs=+-
  One_over_Ns : Gain  Gain=0.0025
  Previous_y : UnitDelay  SampleTime=5e-05  HasFrameUpgradeWarning=on
  y : Outport
  wires:
  x/1 -> Difference/1, Delay_Ns/1
  Delay_Ns/1 -> Difference/2
  Difference/1 -> One_over_Ns/1
  One_over_Ns/1 -> Accumulator/1
  Previous_y/1 -> Accumulator/2
  Accumulator/1 -> y/1, Previous_y/1

== matlab function Fig330L1_THD5_tuned_gridRC2_2wai/MATLAB Function ==
  data: Ualpha input; c1 output; Ubeta input; T input; Ud input; c2 output; c3 output
    function [c1,c2,c3] = SVPWM(Ualpha,Ubeta,T,Ud)
    U1=Ubeta;
    U2=sqrt(3)*Ualpha-Ubeta;
    U3=-Ualpha*sqrt(3)-Ubeta;
    V=0;%扇区
    t1=0;
    t2=0;
    t3=0;
    T11=0;
    T22=0;
    %扇区选择
    if(U1>0)
        A=1;
    else
        A=0;
    end
    if(U2>0)
        B=1;
    else
        B=0;
    end
    if(U3>0)
        C=1;
    else
        C=0;
    end
    N=A+2*B+4*C;
    switch N
        case 1, V=2;
        case 2, V=6;
        case 3, V=1;
        case 4, V=4;
        case 5, V=3;
        case 6, V=5;
    end
   %中间矢量
    X=sqrt(3)*T*Ubeta/Ud;
    Y=(sqrt(3)*Ubeta+3*Ualpha)*T/(2*Ud);
    Z=(sqrt(3)*Ubeta-3*Ualpha)*T/(2*Ud);
    switch V
        case 1
        T11=-Z;T22=X;
        case 2
        T11=Z;T22=Y;
        case 3
        T11=X;T22=-Y;
        case 4
        T11=-X;T22=Z;
        case 5
        T11=-Y;T22=-Z;
        case 6
        T11=Y;T22=-X;
    end
    if(T11+T22>T)
        T1=T11/(T11+T22)*T;
        T2=T22/(T11+T22)*T;
    else
        T1=T11;
        T2=T22;
    end
    ta=(T-T1-T2)/4;
    tb=ta+T1/2;
    tc=tb+T2/2;
    switch V
        case 1
        t1=ta;
        t2=tb;
        t3=tc;
        case 2
        t1=tb;
        t2=ta;
        t3=tc;
        case 3
        t1=tc;
        t2=ta;
        t3=tb;
        case 4
        t1=tc;
        t2=tb;
        t3=ta;
        case 5
        t1=tb;
        t2=tc;
        t3=ta;
        case 6
        t1=ta;
        t2=tc;
        t3=tb;
    end
    c1=t1;
    c2=t2;
    c3=t3;
